simulink model "gm_comm8qamtxrxhdl"  (R2025b)
settings: Solver=FixedStepDiscrete  StartTime=0.0  StopTime=20000*qam_params.symbolPeriod  RelTol=1e-3
PreLoadFcn:
  | qam_params = comm8qamtxrxhdl_init;
InitFcn:
  | qam_params = comm8qamtxrxhdl_init;
undefined symbols (not defined in the file or in its folder): Add, Shift
libraries: simulink x4, hdlsllib x4, dspsigops x2, commchan3 x1, commrflib2 x1, dsphdlmathfun2 x1, dsphdlsigops2 x1, dspmlti4 x1, simulink_need_slupdate x1, hdlmdlgenlib x1, commdigbbndam3 x1, commsequence2 x1
(part 2 of 3)

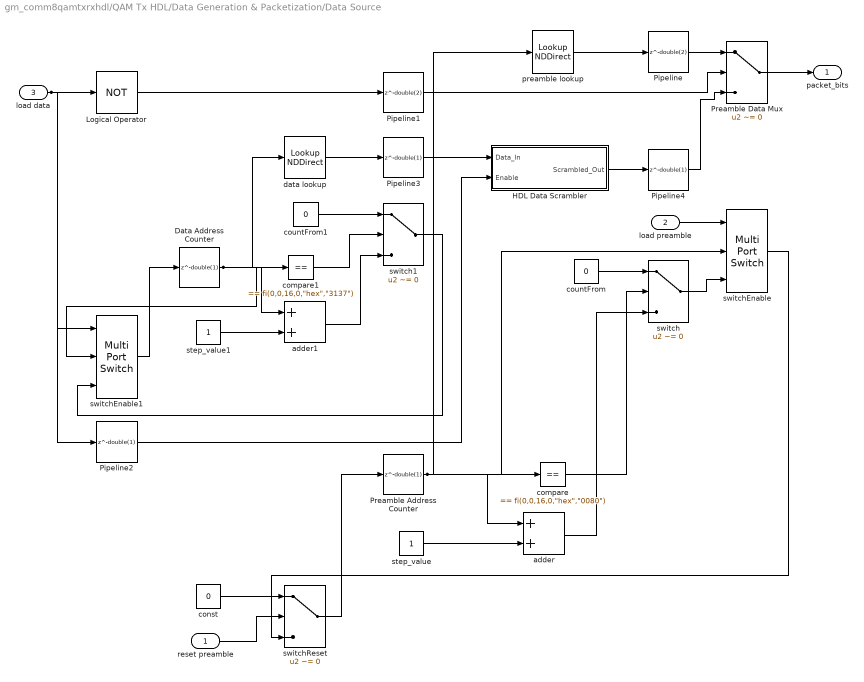
== system gm_comm8qamtxrxhdl/QAM Tx HDL/Data Generation & Packetization/Data Source ==
  reset preamble : Inport  OutDataTypeStr=boolean  PortDimensions=1  SampleTime=3.33333333333333e-07
  load preamble : Inport  Port=2  OutDataTypeStr=boolean  PortDimensions=1  SampleTime=3.33333333333333e-07
  load data : Inport  Port=3  OutDataTypeStr=boolean  PortDimensions=1  SampleTime=3.33333333333333e-07
  Data Address Counter : Delay  DelayLength=double(1)  InitialCondition=0  SampleTime=3.33333333333333e-07
  HDL Data Scrambler : Subsystem
  Logical Operator : Logic  Operator=NOT  Inputs=1  AllPortsSameDT=off  OutDataTypeStr=boolean  SampleTime=3.33333333333333e-07
  Pipeline : Delay  DelayLength=double(2)  InitialCondition=0  SampleTime=3.33333333333333e-07
  Pipeline1 : Delay  DelayLength=double(2)  InitialCondition=0  SampleTime=3.33333333333333e-07
  Pipeline2 : Delay  DelayLength=double(1)  InitialCondition=0  SampleTime=3.33333333333333e-07
  Pipeline3 : Delay  DelayLength=double(1)  InitialCondition=0  SampleTime=3.33333333333333e-07
  Pipeline4 : Delay  DelayLength=double(1)  InitialCondition=0  SampleTime=3.33333333333333e-07
  Preamble Address Counter : Delay  DelayLength=double(1)  InitialCondition=0  SampleTime=3.33333333333333e-07
  Preamble Data Mux : Switch  Criteria=u2 ~= 0  Threshold="fi(0,0,1,0,\"hex\",\"0\")"  OutDataTypeStr=boolean  SampleTime=3.33333333333333e-07  SaturateOnIntegerOverflow=off  InputSameDT=off
  adder : Sum  OutDataTypeStr=uint16  AccumDataTypeStr=uint16  SampleTime=3.33333333333333e-07
  adder1 : Sum  OutDataTypeStr=uint16  AccumDataTypeStr=uint16  SampleTime=3.33333333333333e-07
  compare : simulink/Logic and Bit Operations/Compare To Constant  relop===  const="fi(0,0,16,0,\"hex\",\"0080\")"  OutDataTypeStr=boolean
  compare1 : simulink/Logic and Bit Operations/Compare To Constant  relop===  const="fi(0,0,16,0,\"hex\",\"3137\")"  OutDataTypeStr=boolean
  const : Constant  Value=0  VectorParams1D=off  OutDataTypeStr=uint16  SampleTime=3.33333333333333e-07
  countFrom : Constant  Value=0  VectorParams1D=off  OutDataTypeStr=uint16  SampleTime=3.33333333333333e-07
  countFrom1 : Constant  Value=0  VectorParams1D=off  OutDataTypeStr=uint16  SampleTime=3.33333333333333e-07
  data lookup : LookupNDDirect  NumberOfTableDimensions=1  Table="reshape(double([1;0;0;1;0;0;0;1;1;0;0;1;0;1;1;1;0;1;1;0;0;1;1;0;1;1;0;0;1;1;0;1;1;1;1;0;1;0;0;0;0;1;0;1;0;0;0;0;0;1;1;1;1;1;1;0;0;1;1;1;0;0;0;0;1;0;1;1;0;1;1;0;1;0;0;0;1;1;0;0;0;0;0;1;1;0;0;1;1;0;1;1;1;1;1;1;1;0;0;1;0;0;0;0;0;0;1;1;0;0;0;0;0;1;1;0;0;0;0;0;1;1;0;0;0;0;1;0;0;1;0;0;0;1;1;0;0;1;0;1;1;1;0;1;1;0;0;1;1;0;1;1;0;0;1;1;0;1;1;1;1;0;1;0;0;0;0;1;0;1;0;0;0;0;0;1;1;1;1;1;1;0;0;1;1;1;0;0;0;0;1;0;1;1;0;1;1;0;1;0;0;0;1;1;0;0;0;0;0;1;1;0;0;1;1;0;1;1;1;1;1;1;1;0;0;1;0;0;0;0;0;0;1;1;0;0;0;0;0;1;1;0;0;0;0;0;1;1;0;0;0;1;1;0;0;1;0;0;0;1;1;0;0;1;0;1;1;1;0;1;1;0;0;1;1;0;1;1;0;0;1;1;0;1;1;1;1;0;1;0;0;0;0;1;0;1;0;0;0;0;0;1;1;1;1;1;1;0;0;1;1;1;0;0;0;0;1;0;1;1;0;1;1;0;1;0;0;0;1;1;0;0;0;0;0;1;1;0;0;1;1;0;1;1;1;1;1;1;1;0;0;1;0;0;0;0;0;0;1;1;0;0;0;0;0;1;1;0;0;0;0;0;1;1;0;0;1;0;1;0;0;1;0;0;0;1;1;0;0;1;0;1;1;1;0;1;1;0;0;1;1;0;1;1;0;0;1;1;0;1;1;1;1;0;1;0;0;0;0;1;0;1;0;0;0;0;0;1;1;1;1;1;1;0;0;1;1;1;0;0;0;0;1;0;1;1;0;1;1;0;1;0;0;0;1;1;0;0;0;0;0;1;1;0;0;1;1;0;1;1;1;1;1;1;1;0;0;1;0;0;0;0;0;0;1;1;0;0;0;0;0;1;1;0;0;0;0;0;1;1;0;0;1;1;1;0;0;1;0;0;0;1;1;0;0;1;0;1;1;1;0;1;1;0;0;1;1;0;1;1;0;0;1;1;0;1;1;1;1;0;1;0;0;0;0;1;0;1;0;0;0;0;0;1;1;1;1;1;1;0;0;1;1;1;0;0;0;0;1;0;1;1;0;1;1;0;1;0;0;0;1;1;0;0;0;0;0;1;1;0;0;1;1;0;1;1;1;1;1;1;1;0;0;1;0;0;0;0;0;0;1;1;0;0;0;0;0;1;1;0;0;0;0;0;1;1;0;1;0;0;1;0;0;1;0;0;0;1;1;0;0;1;0;1;1;1;0;1;1;0;0;1;1;0;1;1;0;0;1;1;0;1;1;1;1;0;1;0;0;0;0;1;0;1;0;0;0;0;0;1;1;1;1;1;1;0;0;1;1;1;0;0;0;0;1;0;1;1;0;1;1;0;1;0;0;0;1;1;0;0;0;0;0;1;1;0;0;1;1;0;1;1;1;1;1;1;1;0;0;1;0;0;0;0;0;0;1;1;0;0;0;0;0;1;1;0;0;0;0;0;1;1;0;1;0;1;1;0;0;1;0;0;0;1;1;0;0;1;0;1;1;1;0;1;1;0;0;1;1;0;1;1;0;0;1;1;0;1;1;1;1;0;1;0;0;0;0;1;0;1;0;0;0;0;0;1;1;1;1;1;1;0;0;1;1;1;0;0;0;0;1;0;1;1;0;1;1;0;1;0;0;0;1;1;0;0;0;0;0;1;1;0;0;1;1;0;1;1;1;1;1;1;1;0;0;1;0;0;0;0;0;0;1;1;0;0;0;0;0;1;1;0;0;0;0;0;1;1;0;1;1;0;1;0;0;1;0;0;0;1;1;0;0;1;0;1;1;1;0;1;1;0;0;1;1;0;1;1;0;0;1;1;0;1;1;1;1;0;1;0;0;0;0;1;0;1;0;0;0;0;0;1;1;1;1;1;1;0;0;1;1;1;0;0;0;0;1;0;1;1;0;1;1;0;1;0;0;0;1;1;0;0;0;0;0;1;1;0;0;1;1;0;1;1;1;1;1;1;1;0;0;1;0;0;0;0;0;0;1;1;0;0;0;0;0;1;1;0;0;0;0;0;1;1;0;1;1;1;1;0;0;1;0;0;0;1;1;0;0;1;0;1;1;1;0;1;1;0;0;1;1;0;1;1;0;0;1;1;0;1;1;1;1;0;1;0;0;0;0;1;0;1;0;0;0;0;0;1;1;1;1;1;1;0;0;1;1;1;0;0;0;0;1;0;1;1;0;1;1;0;1;0;0;0;1;1;0;0;0;0;0;1;1;0;0;1;1;0;1;1;1;1;1;1;1;0;0;1;0;0;0;0;0;0;1;1;0;0;0;0;0;1;1;0;0;0;0;0;1;1;1;0;0;0;1;0;0;1;0;0;0;1;1;0;0;1;0;1;1;1;0;1;1;0;0;1;1;0;1;1;0;0;1;1;0;1;1;1;1;0;1;0;0;0;0;1;0;1;0;0;0;0;0;1;1;1;1;1;1;0;0;1;1;1;0;0;0;0;1;0;1;1;0;1;1;0;1;0;0;0;1;1;0;0;0;0;0;1;1;0;0;1;1;0;1;1;1;1;1;1;1;0;0;1;0;0;0;0;0;0;1;1;0;0;0;0;0;1;1;0;0;0;0;0;1;1;1;0;0;1;1;0;0;1;0;0;0;1;1;0;0;1;0;1;1;1;0;1;1;0;0;1;1;0;1;1;0;0;1;1;0;1;1;1;1;0;1;0;0;0;0;1;0;1;0;0;0;0;0;1;1;1;1;1;1;0;0;1;1;1;0;0;0;0;1;0;1;1;0;1;1;0;1;0;0;0;1;1;0;0;0;0;0;1;1;0;0;1;1;0;1;1;1;1;1;1;1;0;0;1;0;0;0;0;0;0;1;1;0;0;0;0;0;1;1;0;0;0;1;0;1;1;0;0;0;0;1;0;0;1;0;0;0;1;1;0;0;1;0;1;1;1;0;1;1;0;0;1;1;0;1;1;0;0;1;1;0;1;1;1;1;0;1;0;0;0;0;1;0;1;0;0;0;0;0;1;1;1;1;1;1;0;0;1;1;1;0;0;0;0;1;0;1;1;0;1;1;0;1;0;0;0;1;1;0;0;0;0;0;1;1;0;0;1;1;0;1;1;1;1;1;1;1;0;0;1;0;0;0;0;0;0;1;1;0;0;0;0;0;1;1;0;0;0;1;0;1;1;0;0;0;1;1;0;0;1;0;0;0;1;1;0;0;1;0;1;1;1;0;1;1;0;0;1;1;0;1;1;0;0;1;1;0;1;1;1;1;0;1;0;0;0;0;1;0;1;0;0;0;0;0;1;1;1;1;1;1;0;0;1;1;1;0;0;0;0;1;0;1;1;0;1;1;0;1;0;0;0;1;1;0;0;0;0;0;1;1;0;0;1;1;0;1;1;1;1;1;1;1;0;0;1;0;0;0;0;0;0;1;1;0;0;0;0;0;1;1;0;0;0;1;0;1;1;0;0;1;0;1;0;0;1;0;0;0;1;1;0;0;1;0;1;1;1;0;1;1;0;0;1;1;0;1;1;0;0;1;1;0;1;1;1;1;0;1;0;0;0;0;1;0;1;0;0;0;0;0;1;1;1;1;1;1;0;0;1;1;1;0;0;0;0;1;0;1;1;0;1;1;0;1;0;0;0;1;1;0;0;0;0;0;1;1;0;0;1;1;0;1;1;1;1;1;1;1;0;0;1;0;0;0;0;0;0;1;1;0;0;0;0;0;1;1;0;0;0;1;0;1;1;0;0;1;1;1;0;0;1;0;0;0;1;1;0;0;1;0;1;1;1;0;1;1;0;0;1;1;0;1;1;0;0;1;1;0;1;1;1;1;0;1;0;0;0;0;1;0;1;0;0;0;0;0;1;1;1;1;1;1;0;0;1;1;1;0;0;0;0;1;0;1;1;0;1;1;0;1;0;0;0;1;1;0;0;0;0;0;1;1;0;0;1;1;0;1;1;1;1;1;1;1;0;0;1;0;0;0;0;0;0;1;1;0;0;0;0;0;1;1;0;0;0;1;0;1;1;0;1;0;0;1;0;0;1;0;0;0;1;1;0;0;1;0;1;1;1;0;1;1;0;0;1;1;0;1;1;0;0;1;1;0;1;1;1;1;0;1;0;0;0;0;1;0;1;0;0;0;0;0;1;1;1;1;1;1;0;0;1;1;1;0;0;0;0;1;0;1;1;0;1;1;0;1;0;0;0;1;1;0;0;0;0;0;1;1;0;0;1;1;0;1;1;1;1;1;1;1;0;0;1;0;0;0;0;0;0;1;1;0 ...(+61538 chars)]), [32768      1])"  DiagnosticForOutOfRangeInput=Error  SampleTime=3.33333333333333e-07  TableDataTypeStr=boolean
  preamble lookup : LookupNDDirect  NumberOfTableDimensions=1  Table="reshape(double([1;0;0;1;0;0;1;0;0;1;0;0;1;0;0;0;0;1;0;0;1;1;0;0;1;0;0;0;0;1;1;0;0;0;0;1;1;0;0;1;0;0;0;0;0;0;0;0;0;0;0;0;0;0;0;0;0;0;0;0;0;0;0;0;0;0;0;0;0;0;0;0;0;0;0;0;0;0;0;0;0;0;0;0;0;0;0;0;0;0;0;0;0;0;0;0;0;0;0;0;0;0;0;0;0;0;0;0;0;0;0;0;0;0;0;0;0;0;0;0;0;0;0;0;0;0;0;0]), [128    1])"  DiagnosticForOutOfRangeInput=Error  SampleTime=3.33333333333333e-07  TableDataTypeStr=boolean
  step_value : Constant  VectorParams1D=off  OutDataTypeStr=uint16  SampleTime=3.33333333333333e-07
  step_value1 : Constant  VectorParams1D=off  OutDataTypeStr=uint16  SampleTime=3.33333333333333e-07
  switch : Switch  Criteria=u2 ~= 0  Threshold="fi(0,0,1,0,\"hex\",\"0\")"  OutDataTypeStr=uint16  SampleTime=3.33333333333333e-07  SaturateOnIntegerOverflow=off  InputSameDT=off
  switch1 : Switch  Criteria=u2 ~= 0  Threshold="fi(0,0,1,0,\"hex\",\"0\")"  OutDataTypeStr=uint16  SampleTime=3.33333333333333e-07  SaturateOnIntegerOverflow=off  InputSameDT=off
  switchEnable : MultiPortSwitch  DataPortOrder=Zero-based contiguous  Inputs=2  DiagnosticForDefault=None  zeroidx=on  OutDataTypeStr=uint16  SampleTime=3.33333333333333e-07  SaturateOnIntegerOverflow=off  InputSameDT=off
  switchEnable1 : MultiPortSwitch  DataPortOrder=Zero-based contiguous  Inputs=2  DiagnosticForDefault=None  zeroidx=on  OutDataTypeStr=uint16  SampleTime=3.33333333333333e-07  SaturateOnIntegerOverflow=off  InputSameDT=off
  switchReset : Switch  Criteria=u2 ~= 0  Threshold="fi(0,0,1,0,\"hex\",\"0\")"  OutDataTypeStr=uint16  SampleTime=3.33333333333333e-07  SaturateOnIntegerOverflow=off  InputSameDT=off
  packet_bits : Outport  SampleTime=3.33333333333333e-07  VectorParamsAs1DForOutWhenUnconnected=off
  wires:
  load data/1 -> Pipeline2/1, Logical Operator/1, switchEnable1/1
  Logical Operator/1 -> Pipeline1/1
  switchEnable1/1 -> Data Address Counter/1
  step_value1/1 -> adder1/2
  Pipeline2/1 -> HDL Data Scrambler/2(Enable)
  reset preamble/1 -> switchReset/2
  Data Address Counter/1 -> switchEnable1/2, data lookup/1, compare1/1, adder1/1
  const/1 -> switchReset/1
  switchReset/1 -> Preamble Address Counter/1
  data lookup/1 -> Pipeline3/1
  countFrom1/1 -> switch1/1
  compare1/1 -> switch1/2
  adder1/1 -> switch1/3
  Pipeline1/1 -> Preamble Data Mux/2
  Pipeline3/1 -> HDL Data Scrambler/1(Data_In)
  HDL Data Scrambler/1(Scrambled_Out) -> Pipeline4/1
  switch1/1 -> switchEnable1/3
  preamble lookup/1 -> Pipeline/1
  Preamble Address Counter/1 -> switchEnable/2, preamble lookup/1, compare/1, adder/1
  step_value/1 -> adder/2
  countFrom/1 -> switch/1
  compare/1 -> switch/2
  adder/1 -> switch/3
  Pipeline/1 -> Preamble Data Mux/1
  switchEnable/1 -> switchReset/3
  Pipeline4/1 -> Preamble Data Mux/3
  load preamble/1 -> switchEnable/1
  switch/1 -> switchEnable/3
  Preamble Data Mux/1 -> packet_bits/1
